simulink model "LKM_AW_Core_F405"  (R2026b)
settings: Solver=FixedStepDiscrete  FixedStep=0.01  EnableMultiTasking=on
model workspace (MAT data in the model file):
  K_achieved_core = [1  1  1  1; -0.0742462128401  -0.0742462128401  0.0742462128401  0.0742462128401; -0.0742462128401  0.0742462128401  -0.0742462128401  0.0742462128401]
settings OptimizationCC: DefaultParameterBehavior=Inlined  DifferentSizesBufferReuse=on  EfficientTunableParamExpr=on  EnhancedBackFolding=on  MaxStackSize=512  OptimizationCustomize=off  OptimizeBlockOrder=speed  PassReuseOutputArgsAs=Individual arguments  RemoveInternalMemoryZeroInit=on  RemoveRootLevelIOMemoryZeroInit=on
settings DebuggingCC: ParameterTunabilityLossMsg=error
settings HardwareCC: ProdHWDeviceType=ARM Compatible->ARM Cortex-M  ProdLargestAtomicFloat=Double  ProdLargestAtomicInteger=Long  ProdLongLongMode=on
settings SFSimCC: MATLABDynamicMemAlloc=off
settings RTWCC: BuildConfiguration=Faster Runs  DataTypeReplacement=CDataTypesFixedWidth  Description=Embedded Coder  HardwareBoard=STM32F4xx Based  SystemTargetFile=ert.tlc  TLCOptions=-aInlineSetEventsForThisBaseRateFcn=TLC_FALSE -aSuppressMultiTaskScheduler=TLC_FALSE -aRateBasedStepFcn=1  TemplateMakefile=ert_default_tmf  Toolchain=GNU Tools for STM32
settings CodeAppCC: ForceParamTrailComments=on  IgnoreCustomStorageClasses=off  InsertBlockDesc=on  OperatorAnnotations=on  SFDataObjDesc=on  SimulinkDataObjDesc=on
settings ERTTargetCC: CodeReplacementLibrary=ARM Cortex-M  CombineSignalStateStructs=on  ExtModeIntrfLevel=Level2 - Open  ExtModeMexFile=ext_xcp  ExtModeStaticAlloc=on  MaxIdInt16=INT16_MAX  MaxIdInt32=INT32_MAX  MaxIdInt64=INT64_MAX  MaxIdInt8=INT8_MAX  MaxIdUint16=UINT16_MAX  MaxIdUint32=UINT32_MAX  MaxIdUint64=UINT64_MAX  MaxIdUint8=UINT8_MAX  MinIdInt16=INT16_MIN  MinIdInt32=INT32_MIN  MinIdInt64=INT64_MIN  MinIdInt8=INT8_MIN

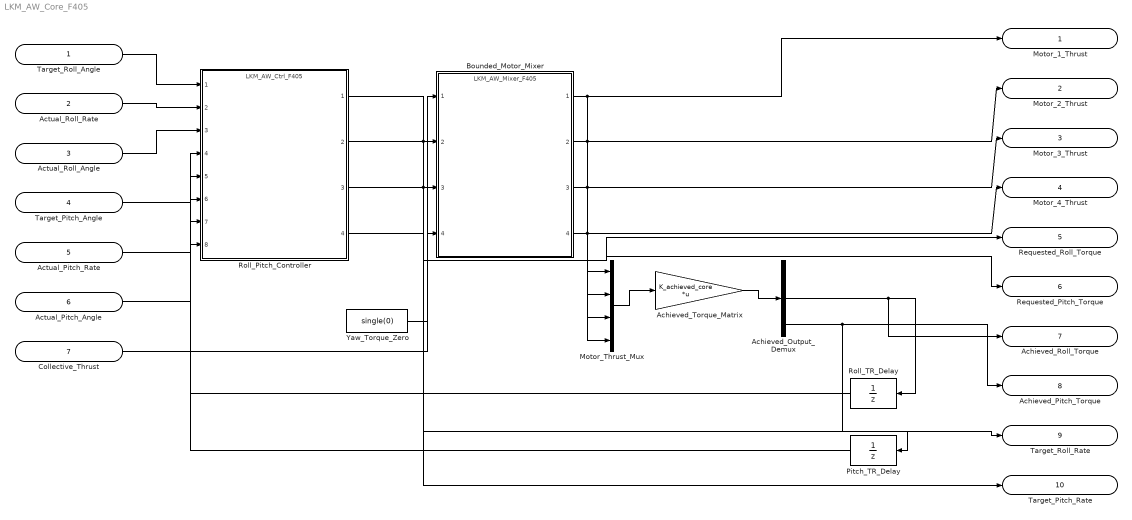
== system LKM_AW_Core_F405 ==
  Target_Roll_Angle : Inport  OutDataTypeStr=single  SampleTime=0.01
  Actual_Roll_Rate : Inport  Port=2  OutDataTypeStr=single  SampleTime=0.01
  Actual_Roll_Angle : Inport  Port=3  OutDataTypeStr=single  SampleTime=0.01
  Target_Pitch_Angle : Inport  Port=4  OutDataTypeStr=single  SampleTime=0.01
  Actual_Pitch_Rate : Inport  Port=5  OutDataTypeStr=single  SampleTime=0.01
  Actual_Pitch_Angle : Inport  Port=6  OutDataTypeStr=single  SampleTime=0.01
  Collective_Thrust : Inport  Port=7  OutDataTypeStr=single  SampleTime=0.01
  Achieved_Output_Demux : Demux  Outputs=3
  Achieved_Torque_Matrix : Gain  Gain=K_achieved_core  Multiplication=Matrix(K*u)
  Bounded_Motor_Mixer : ModelReference  ModelNameDialog=LKM_AW_Mixer_F405  SimulationMode=Normal  ModelReferenceVersion=1.11
  Motor_Thrust_Mux : Mux
  Pitch_TR_Delay : UnitDelay  InitialCondition=single(0)  SampleTime=0.01
  Roll_Pitch_Controller : ModelReference  ModelNameDialog=LKM_AW_Ctrl_F405  SimulationMode=Normal  ModelReferenceVersion=1.25
  Roll_TR_Delay : UnitDelay  InitialCondition=single(0)  SampleTime=0.01
  Yaw_Torque_Zero : Constant  Value=single(0)  OutDataTypeStr=single
  Motor_1_Thrust : Outport
  Motor_2_Thrust : Outport  Port=2
  Motor_3_Thrust : Outport  Port=3
  Motor_4_Thrust : Outport  Port=4
  Requested_Roll_Torque : Outport  Port=5
  Requested_Pitch_Torque : Outport  Port=6
  Achieved_Roll_Torque : Outport  Port=7
  Achieved_Pitch_Torque : Outport  Port=8
  Target_Roll_Rate : Outport  Port=9
  Target_Pitch_Rate : Outport  Port=10
  wires:
  Target_Roll_Angle/1 -> Roll_Pitch_Controller/1
  Actual_Roll_Rate/1 -> Roll_Pitch_Controller/2
  Actual_Roll_Angle/1 -> Roll_Pitch_Controller/3
  Target_Pitch_Angle/1 -> Roll_Pitch_Controller/4
  Actual_Pitch_Rate/1 -> Roll_Pitch_Controller/5
  Actual_Pitch_Angle/1 -> Roll_Pitch_Controller/6
  Collective_Thrust/1 -> Bounded_Motor_Mixer/1
  Yaw_Torque_Zero/1 -> Bounded_Motor_Mixer/4
  Roll_Pitch_Controller/1 -> Bounded_Motor_Mixer/2, Requested_Roll_Torque/1
  Roll_Pitch_Controller/3 -> Bounded_Motor_Mixer/3, Requested_Pitch_Torque/1
  Bounded_Motor_Mixer/1 -> Motor_1_Thrust/1, Motor_Thrust_Mux/1
  Bounded_Motor_Mixer/2 -> Motor_2_Thrust/1, Motor_Thrust_Mux/2
  Bounded_Motor_Mixer/3 -> Motor_3_Thrust/1, Motor_Thrust_Mux/3
  Bounded_Motor_Mixer/4 -> Motor_4_Thrust/1, Motor_Thrust_Mux/4
  Motor_Thrust_Mux/1 -> Achieved_Torque_Matrix/1
  Achieved_Torque_Matrix/1 -> Achieved_Output_Demux/1
  Achieved_Output_Demux/2 -> Roll_TR_Delay/1, Achieved_Roll_Torque/1
  Roll_TR_Delay/1 -> Roll_Pitch_Controller/7
  Achieved_Output_Demux/3 -> Pitch_TR_Delay/1, Achieved_Pitch_Torque/1
  Pitch_TR_Delay/1 -> Roll_Pitch_Controller/8
  Roll_Pitch_Controller/2 -> Target_Roll_Rate/1
  Roll_Pitch_Controller/4 -> Target_Pitch_Rate/1
